simulink model "nlMPC_simulation_NN_obs"  (R2026b)
settings: Solver=FixedStepAuto  StopTime=50*Ts  FixedStep=Ts
values from neighbouring files (symbols this model uses):
  bf = evalin('base','bf')    [EKF_MeasurementFcn_coder_ext.m]    (also in RNN_syst.m = [-0.9006506])
  bxu = evalin('base','bxu')    [EKF_StateTransitionFcn_coder_ext.m]    (also in RNN_syst.m = [-0.5022973 0.41583735 0.32208467 -0.12734303 -0.56159854 0.)
  coef_input = evalin('base','coef_input')    [EKF_StateTransitionFcn_coder_ext.m]
  N = 20    [MPC.m]    (also in MPC_NN_ident_2A_obs.m)
  nx = length(bxu)    [RNN_syst.m]
  T0 = evalin('base','T0')    [EKF_MeasurementFcn_coder_ext.m]
  Ts = 0.00001    (= 1e-05)    [random_init.m]
  Wf = evalin('base','Wf')    [EKF_MeasurementFcn_coder_ext.m]    (also in RNN_syst.m = [0.77021164 -1.0041683 -0.89421856 -0.74259216 0.9288221 -0.)
  Wu = evalin('base','Wu')    [EKF_StateTransitionFcn_coder_ext.m]    (also in RNN_syst.m = [0.40815163; 0.057077326; -0.20906386; -0.058028016; 0.01622)
  Wx = evalin('base','Wx')    [EKF_StateTransitionFcn_coder_ext.m]    (also in RNN_syst.m = [0.093657404 -0.03755194 -0.1360607 -0.106877 0.15790185 -0.)
  y_span = evalin('base','y_span')    [EKF_MeasurementFcn_coder_ext.m]
undefined symbols (not defined in the file or in its folder): A, Cth, emissivity, h, Ta
libraries: mpclib x2, sharedTrackingLibrary x2, simulink x1
settings Model: Creator=Max  LastModifiedBy=chalqua
settings OptimizationCC: ReuseModelBlockBuffer=off
settings DebuggingCC: UnderSpecifiedDimensionMsg=warning

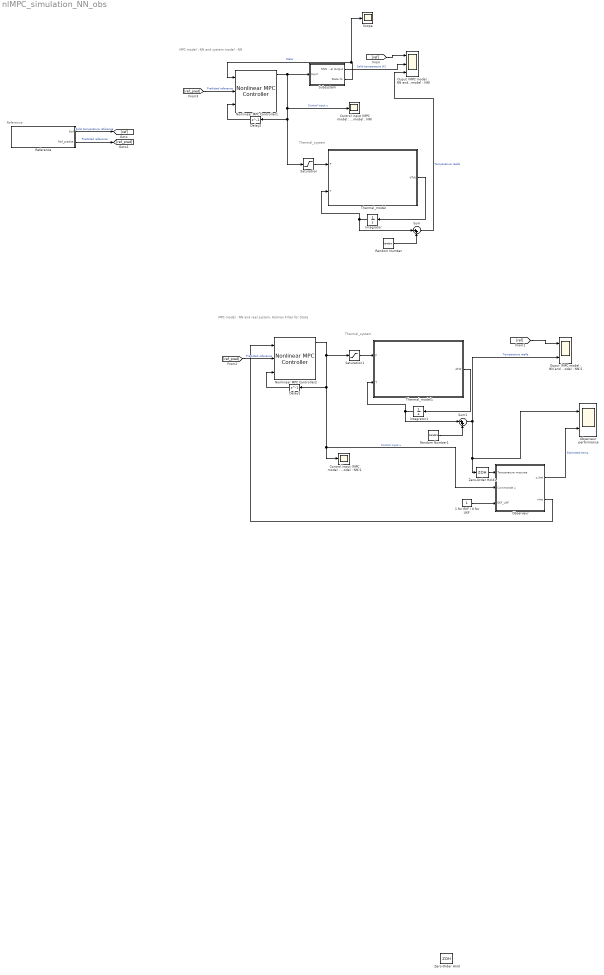
== system nlMPC_simulation_NN_obs ==
  note: MPC model : NN and system model : NN
  note: Reference
  note: Thermal_system
  note: Thermal_system
  note: MPC model : NN and real system, Kalman Filter for State
  1 for EKF / 0 for UKF : Constant
  "Control input (MPC model : NN and system model : NN)" : Scope
      settings: ActiveDisplayYMinimum=-6.00306055711863  ActiveDisplayYMaximum=22.889228950790958  DataLoggingVariableName=ScopeData4
  "Control input (MPC model : NN and system model : NN)1" : Scope
      settings: ActiveDisplayYMinimum=-6.00306055711863  ActiveDisplayYMaximum=22.889228950790958
  Delay1 : Delay  DelayLength=1  InitialCondition=0  SampleTime=Ts
  Delay2 : Delay  DelayLength=1  InitialCondition=0  SampleTime=Ts
  Integrator : Integrator  InitialCondition=T0
  Integrator1 : Integrator  InitialCondition=T0
  Nonlinear MPC Controller1 : mpclib/Nonlinear MPC Controller  SCDEnableBlockLinearizationSpecification=on  nlmpcobj=nlmpc_nn  md_enabled=off  mvtarget_enabled=off  param_enabled=off  cost_enabled=on  mvseq_enabled=on  stateseq_enabled=on  ovseq_enabled=on  slack_enabled=off  status_enabled=on  ov_min=off  ov_max=off  mv_min=off  mv_max=off  mvrate_min=off  mvrate_max=off  state_min=off  state_max=off  ov_weight=off  mv_weight=off  mvrate_weight=off  ecr_weight=off  nlp_initialize=off  BlockDataType=double  UseObjectTs=on  UseMEX=off
  Nonlinear MPC Controller2 : mpclib/Nonlinear MPC Controller  SCDEnableBlockLinearizationSpecification=on  nlmpcobj=nlmpc_nn  md_enabled=off  mvtarget_enabled=off  param_enabled=off  cost_enabled=on  mvseq_enabled=on  stateseq_enabled=on  ovseq_enabled=on  slack_enabled=off  status_enabled=on  ov_min=off  ov_max=off  mv_min=off  mv_max=off  mvrate_min=off  mvrate_max=off  state_min=off  state_max=off  ov_weight=off  mv_weight=off  mvrate_weight=off  ecr_weight=off  nlp_initialize=off  BlockDataType=double  UseObjectTs=on  UseMEX=off
  Observeur : Subsystem
  Observeur performance : Scope  NumInputPorts=2
      settings: ActiveDisplayYMinimum=271.23494170506268  ActiveDisplayYMaximum=414.42853112318659  DataLoggingVariableName=ScopeData3
  "Ouput (MPC model : NN and system model : NN)" : Scope  NumInputPorts=3
      settings: SampleTime=Ts  ActiveDisplayYMinimum=276.4435919871114  ActiveDisplayYMaximum=413.72848977920984  DataLoggingVariableName=output_simulink
  "Ouput (MPC model : NN and system model : NN)1" : Scope  NumInputPorts=2
      settings: SampleTime=Ts  ActiveDisplayYMinimum=276.4435919871114  ActiveDisplayYMaximum=413.72848977920984  DataLoggingVariableName=output_simulink1
  Random Number : RandomNumber  Variance=0.02  Seed=52142  SampleTime=190
  Random Number1 : RandomNumber  Variance=0.02  Seed=52142  SampleTime=190
  Reference : Subsystem
  Saturation : Saturate  UpperLimit=20  LowerLimit=-20
  Saturation1 : Saturate  UpperLimit=20  LowerLimit=-20
  Scope : Scope
      settings: ActiveDisplayYMinimum=-1.018053850942551  ActiveDisplayYMaximum=0.73269388464727869
  Subsystem : Subsystem
  Sum : Sum  Inputs=|++
  Sum1 : Sum  Inputs=|++
  Thermal_model : MATLAB Function  TreatAsAtomicUnit=on
  Thermal_model1 : MATLAB Function  TreatAsAtomicUnit=on
  Zero-Order Hold : ZeroOrderHold  SampleTime=-1
  Zero-Order Hold1 : ZeroOrderHold  SampleTime=Ts
  wires:
  Subsystem/1(RNN Model Output) -> "Ouput (MPC model : NN and system model : NN)"/2  "Solid temperature [K]"
  Delay2/1 -> Nonlinear MPC Controller1/3
  Nonlinear MPC Controller1/1 -> Subsystem/1(Input), "Control input (MPC model : NN and system model : NN)"/1, Saturation/1, Delay2/1  "Control input u"
  Subsystem/2(State hk) -> Scope/1, Nonlinear MPC Controller1/1  "State"
  [ref_pred] -> Nonlinear MPC Controller1/2  "Predicted reference"
  Reference/1(Ref) -> [ref]  "Solid temperature reference"
  Reference/2(Ref_predite) -> [ref_pred]  "Predicted reference"
  [ref] -> "Ouput (MPC model : NN and system model : NN)"/1
  Saturation/1 -> Thermal_model/1(P)
  Thermal_model/1(dTdt) -> Integrator/1
  Sum/1 -> "Ouput (MPC model : NN and system model : NN)"/3  "Température réelle"
  Integrator/1 -> Sum/1, Thermal_model/2(T)
  Random Number/1 -> Sum/2
  1 for EKF / 0 for UKF/1 -> Observeur/3(EKF_UKF)
  Random Number1/1 -> Sum1/2
  Nonlinear MPC Controller2/1 -> Delay1/1, "Control input (MPC model : NN and system model : NN)1"/1, Observeur/2(Commande u), Saturation1/1  "Control input u"
  Saturation1/1 -> Thermal_model1/1(P)
  [ref] -> "Ouput (MPC model : NN and system model : NN)1"/1
  Delay1/1 -> Nonlinear MPC Controller2/3
  [ref_pred] -> Nonlinear MPC Controller2/2  "Predicted reference"
  Integrator1/1 -> Sum1/1, Thermal_model1/2(T)
  Sum1/1 -> Zero-Order Hold1/1, Observeur performance/1, "Ouput (MPC model : NN and system model : NN)1"/2  "Température réelle"
  Thermal_model1/1(dTdt) -> Integrator1/1
  Observeur/1(y_hat) -> Observeur performance/2  "Estimated temp"
  Observeur/2(xhat) -> Nonlinear MPC Controller2/1
  Zero-Order Hold1/1 -> Observeur/1(Temperature mesurée)

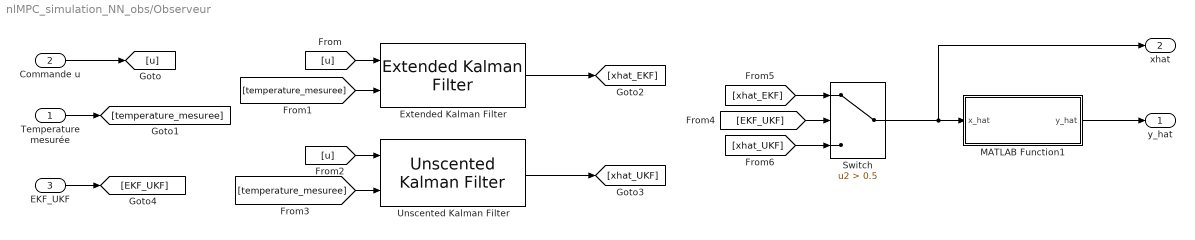
== system nlMPC_simulation_NN_obs/Observeur ==
  Temperature mesurée : Inport
  Commande u : Inport  Port=2
  EKF_UKF : Inport  Port=3
  Extended Kalman Filter : sharedTrackingLibrary/Extended Kalman Filter  StateTransitionFcn=EKF_StateTransitionFcn  HasStateTransitionJacobianFcn=off  HasAdditiveProcessNoise=Additive  ProcessNoise=1  HasTimeVaryingProcessNoise=off  HasStateTransitionFcnExtraArgument=1  InitialState=ones(nx,1)*T0  InitialStateCovariance=1  MeasurementFcn1=EKF_MeasurementFcn  HasMeasurementJacobianFcn1=off  HasMeasurementEnablePort1=off  HasAdditiveMeasurementNoise1=Additive  MeasurementNoise1=1  HasTimeVaryingMeasurementNoise1=off  HasMeasurementFcnExtraArgument1=0  HasMeasurementWrapping1=off  MeasurementFcn2=myMeasurementFcn  HasMeasurementJacobianFcn2=off  HasMeasurementEnablePort2=off  HasAdditiveMeasurementNoise2=Additive  MeasurementNoise2=1  HasTimeVaryingMeasurementNoise2=off  HasMeasurementFcnExtraArgument2=0  HasMeasurementWrapping2=off  MeasurementFcn3=myMeasurementFcn  HasMeasurementJacobianFcn3=off  HasMeasurementEnablePort3=off  HasAdditiveMeasurementNoise3=Additive  MeasurementNoise3=1  HasTimeVaryingMeasurementNoise3=off  HasMeasurementFcnExtraArgument3=0  HasMeasurementWrapping3=off  MeasurementFcn4=myMeasurementFcn  HasMeasurementJacobianFcn4=off  HasMeasurementEnablePort4=off  HasAdditiveMeasurementNoise4=Additive  MeasurementNoise4=1  HasTimeVaryingMeasurementNoise4=off  HasMeasurementFcnExtraArgument4=0  HasMeasurementWrapping4=off  MeasurementFcn5=myMeasurementFcn  HasMeasurementJacobianFcn5=off  HasMeasurementEnablePort5=off  HasAdditiveMeasurementNoise5=Additive  MeasurementNoise5=1  HasTimeVaryingMeasurementNoise5=off  HasMeasurementFcnExtraArgument5=0  HasMeasurementWrapping5=off  EnableMultirate=off  StateTransitionFcnSampleTime=1  MeasurementFcn1SampleTime=1  MeasurementFcn2SampleTime=1  MeasurementFcn3SampleTime=1  MeasurementFcn4SampleTime=1  MeasurementFcn5SampleTime=1  UseCurrentEstimator=on  OutputStateCovariance=off  DataType=double  SampleTime=Ts  NumberOfMeasurements=1
  MATLAB Function1 : MATLAB Function  TreatAsAtomicUnit=on
  Switch : Switch  Criteria=u2 > Threshold  Threshold=0.5  SaturateOnIntegerOverflow=off  InputSameDT=off
  Unscented Kalman Filter : sharedTrackingLibrary/Unscented Kalman Filter  StateTransitionFcn=EKF_StateTransitionFcn  HasAdditiveProcessNoise=Additive  ProcessNoise=1  HasTimeVaryingProcessNoise=off  HasStateTransitionFcnExtraArgument=1  InitialState=ones(nx,1)*T0  InitialStateCovariance=1  Alpha=1e-3  Beta=2  Kappa=0  MeasurementFcn1=EKF_MeasurementFcn  HasMeasurementEnablePort1=off  HasAdditiveMeasurementNoise1=Additive  MeasurementNoise1=1  HasTimeVaryingMeasurementNoise1=off  HasMeasurementFcnExtraArgument1=0  HasMeasurementWrapping1=off  MeasurementFcn2=myMeasurementFcn  HasMeasurementEnablePort2=off  HasAdditiveMeasurementNoise2=Additive  MeasurementNoise2=1  HasTimeVaryingMeasurementNoise2=off  HasMeasurementFcnExtraArgument2=0  HasMeasurementWrapping2=off  MeasurementFcn3=myMeasurementFcn  HasMeasurementEnablePort3=off  HasAdditiveMeasurementNoise3=Additive  MeasurementNoise3=1  HasTimeVaryingMeasurementNoise3=off  HasMeasurementFcnExtraArgument3=0  HasMeasurementWrapping3=off  MeasurementFcn4=myMeasurementFcn  HasMeasurementEnablePort4=off  HasAdditiveMeasurementNoise4=Additive  MeasurementNoise4=1  HasTimeVaryingMeasurementNoise4=off  HasMeasurementFcnExtraArgument4=0  HasMeasurementWrapping4=off  MeasurementFcn5=myMeasurementFcn  HasMeasurementEnablePort5=off  HasAdditiveMeasurementNoise5=Additive  MeasurementNoise5=1  HasTimeVaryingMeasurementNoise5=off  HasMeasurementFcnExtraArgument5=0  HasMeasurementWrapping5=off  EnableMultirate=off  StateTransitionFcnSampleTime=1  MeasurementFcn1SampleTime=1  MeasurementFcn2SampleTime=1  MeasurementFcn3SampleTime=1  MeasurementFcn4SampleTime=1  MeasurementFcn5SampleTime=1  UseCurrentEstimator=on  OutputStateCovariance=off  DataType=double  SampleTime=Ts  NumberOfMeasurements=1
  y_hat : Outport
  xhat : Outport  Port=2
  wires:
  MATLAB Function1/1(y_hat) -> y_hat/1
  Unscented Kalman Filter/1 -> [xhat_UKF]
  [u] -> Extended Kalman Filter/1
  Commande u/1 -> [u]
  Temperature mesurée/1 -> [temperature_mesuree]
  [temperature_mesuree] -> Extended Kalman Filter/2
  [u] -> Unscented Kalman Filter/1
  [temperature_mesuree] -> Unscented Kalman Filter/2
  Extended Kalman Filter/1 -> [xhat_EKF]
  EKF_UKF/1 -> [EKF_UKF]
  [EKF_UKF] -> Switch/2
  [xhat_EKF] -> Switch/1
  [xhat_UKF] -> Switch/3
  Switch/1 -> MATLAB Function1/1(x_hat), xhat/1

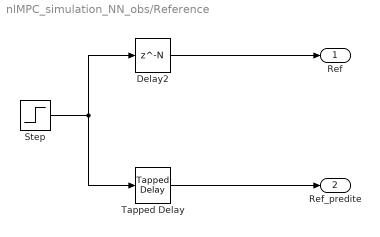
== system nlMPC_simulation_NN_obs/Reference ==
  Delay2 : Delay  DelayLength=N  InitialCondition=T0  SampleTime=Ts
  Step : Step  Time=3  InitialValue=T0  FinalValue=400  SampleTime=Ts
  Tapped Delay : simulink/Discrete/Tapped Delay  vinit=ones(N-1,1)*T0;  samptime=Ts  NumDelays=N-1  DelayOrder=Oldest  includeCurrent=on
  Ref : Outport
  Ref_predite : Outport  Port=2
  wires:
  Step/1 -> Tapped Delay/1, Delay2/1
  Tapped Delay/1 -> Ref_predite/1
  Delay2/1 -> Ref/1

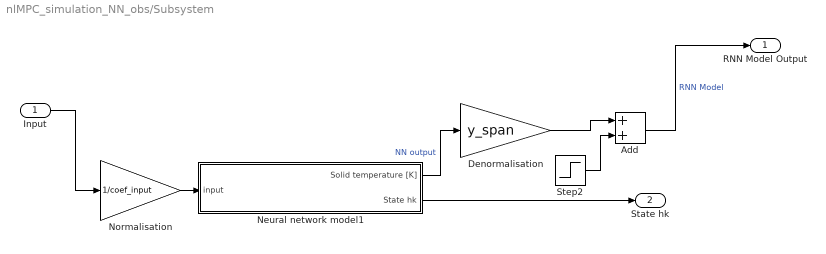
== system nlMPC_simulation_NN_obs/Subsystem ==
  Input : Inport
  Add : Sum
  Denormalisation : Gain  Gain=y_span
  Neural network model1 : Subsystem
  Normalisation : Gain  Gain=1/coef_input
  Step2 : Step  Time=0  InitialValue=T0  FinalValue=T0  SampleTime=0
  RNN Model Output : Outport
  State hk : Outport  Port=2
  wires:
  Input/1 -> Normalisation/1
  Neural network model1/2(State hk) -> State hk/1
  Add/1 -> RNN Model Output/1  "RNN Model"
  Normalisation/1 -> Neural network model1/1(input)
  Neural network model1/1(Solid temperature [K]) -> Denormalisation/1  "NN output"
  Step2/1 -> Add/2
  Denormalisation/1 -> Add/1

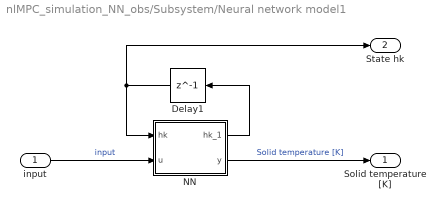
== system nlMPC_simulation_NN_obs/Subsystem/Neural network model1 ==
  input : Inport
  Delay1 : Delay  DelayLength=1  InitialCondition=zeros(nx,1)  SampleTime=Ts
  NN : MATLAB Function  TreatAsAtomicUnit=on  SystemSampleTime=Ts
  Solid temperature [K] : Outport
  State hk : Outport  Port=2
  wires:
  Delay1/1 -> NN/1(hk), State hk/1
  NN/1(hk_1) -> Delay1/1
  input/1 -> NN/2(u)  "input"
  NN/2(y) -> Solid temperature [K]/1  "Solid temperature [K]"

== matlab function nlMPC_simulation_NN_obs/Thermal_model ==
  data: P input; dTdt output; T input; emissivity parameter; Ta parameter; A parameter; h parameter; Cth parameter
function dTdt = thermal_model(P, T, emissivity, Ta, A, h, Cth)
    %#codegen
    % Continuous-time nonlinear thermal model.
    %
    % Inputs:
    %   P          - Heating power [W]
    %   T          - Solid temperature [K]
    %   Cth        - Thermal capacitance [J/K]
    %   h          - Convective heat transfer coefficient [W/(m^2 K)]
    %   A          - Heat exchange surface area [m^2]
    %   emissivity - Surface emissivity [-]
    %   Ta         - Ambient temperature [K]
    %
    % Output:
    %   dTdt       - Temperature derivative [K/s]
    %
    % Model assumptions:
    %   - Uniform temperature inside the solid
    %   - Constant ambient temperature
    %   - Constant physical parameters
    
    % Stefan-Boltzmann constant [W/(m^2 K^4)]
    sigma = 5.670374419e-8;
    
    % Convective heat losses [W]
    Qconv = h * A * (T - Ta);
    
    % Radiative heat losses [W]
    Qrad = emissivity * sigma * A * (T^4 - Ta^4);
    
    % Compute the temperature derivative [K/s]
    dTdt = (P - Qconv - Qrad) / Cth;

end

== matlab function nlMPC_simulation_NN_obs/Observeur/MATLAB Function1 ==
  data: x_hat input; y_hat output
function y_hat = fcn(x_hat)

    y_hat = EKF_MeasurementFcn(x_hat);

end

== matlab function nlMPC_simulation_NN_obs/Thermal_model1 ==
  data: P input; dTdt output; T input; emissivity parameter; Ta parameter; A parameter; h parameter; Cth parameter
function dTdt = thermal_model(P, T, emissivity, Ta, A, h, Cth)
    %#codegen
    % Continuous-time nonlinear thermal model.
    %
    % Inputs:
    %   P          - Heating power [W]
    %   T          - Solid temperature [K]
    %   Cth        - Thermal capacitance [J/K]
    %   h          - Convective heat transfer coefficient [W/(m^2 K)]
    %   A          - Heat exchange surface area [m^2]
    %   emissivity - Surface emissivity [-]
    %   Ta         - Ambient temperature [K]
    %
    % Output:
    %   dTdt       - Temperature derivative [K/s]
    %
    % Model assumptions:
    %   - Uniform temperature inside the solid
    %   - Constant ambient temperature
    %   - Constant physical parameters
    
    % Stefan-Boltzmann constant [W/(m^2 K^4)]
    sigma = 5.670374419e-8;
    
    % Convective heat losses [W]
    Qconv = h * A * (T - Ta);
    
    % Radiative heat losses [W]
    Qrad = emissivity * sigma * A * (T^4 - Ta^4);
    
    % Compute the temperature derivative [K/s]
    dTdt = (P - Qconv - Qrad) / Cth;

end

== matlab function nlMPC_simulation_NN_obs/Subsystem/Neural network model1/NN ==
  data: hk input; u input; hk_1 output; y output; Wx parameter; Wf parameter; bxu parameter; bf parameter; Wu parameter
function [hk_1,y] = fcn(hk,u,Wx, Wf, bxu, bf, Wu)

    % Wrapper function for the neural network submarine model
    % Calls the 'thermal_model_NN' function to update hidden state and output
    % Inputs:
    %   hk  - current hidden state vector
    %   u   - control input
    %   Wx  - hidden-to-hidden weight matrix
    %   Wf  - hidden-to-output weight vector
    %   bxu - hidden layer bias vector
    %   bf  - output layer bias
    %   Wu  - input-to-hidden weight vector
    % Outputs:
    %   hk_1 - updated hidden state at next time step
    %   y    - output of the neural network

    [hk_1,y] = thermal_model_NN(hk,u,Wx, Wf, bxu, bf, Wu);
    
end
